simulink model "HFMA_4B_1_5_9_13"  (R2026b)
settings: Solver=FixedStepDiscrete  StopTime=stopTime  FixedStep=Ts
PreLoadFcn:
  | load('a_luts.mat')
values from neighbouring files (symbols this model uses):
  cosLUT = [1 1 1 1 1 1 1 1 1 1 1 1 ... (640 elements, 16x40)]    [iq_luts.mat]
  k_avg = 10    [Simulink_DOA_Test.m]    (also in collect_ranges.m; optimised_error_code.m)
  sinLUT = [0 0 0 0 0 0 0 0 0 0 0 0 ... (640 elements, 16x40)]    [iq_luts.mat]
  Ts = 1/8000    (= 0.000125)    [Simulink_DOA_Test.m]    (also in collect_ranges.m; optimised_error_code.m)
undefined symbols (not defined in the file or in its folder): a2_Im, a2_Re, a3_Im, a3_Re, NumBits1, NumBits2, Slope1, Slope2
libraries: hdlsllib x4, sl_signal_attributes x2
(part 2 of 6)

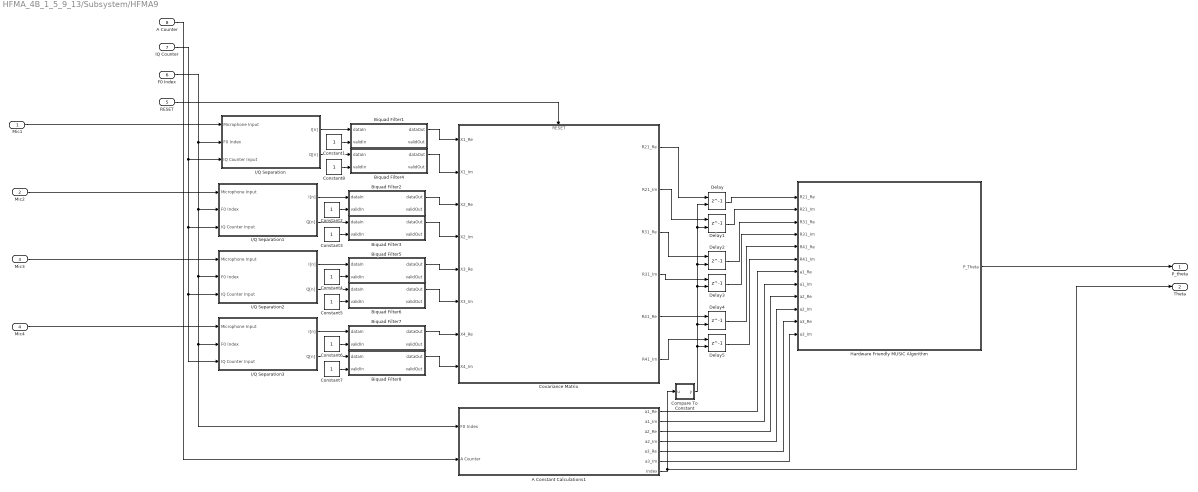
== system HFMA_4B_1_5_9_13/Subsystem/HFMA9 ==
  Mic1 : Inport
  Mic2 : Inport  Port=2
  Mic3 : Inport  Port=3
  Mic4 : Inport  Port=4
  RESET : Inport  Port=5
  F0 Index : Inport  Port=6
  IQ Counter : Inport  Port=7
  A Counter : Inport  Port=8
  A Constant Calculations1 : Subsystem
  Biquad Filter1 : Subsystem
  Biquad Filter2 : Subsystem
  Biquad Filter3 : Subsystem
  Biquad Filter4 : Subsystem
  Biquad Filter5 : Subsystem
  Biquad Filter6 : Subsystem
  Biquad Filter7 : Subsystem
  Biquad Filter8 : Subsystem
  Compare To Constant : Subsystem  mask(Compare To Constant){relop===, const=180, OutDataTypeStr=boolean, ZeroCross=on}
      mask prompts: relop "Simulink:masks:Operator_MP"; const "Simulink:masks:ConstantValue_MP"; OutDataTypeStr "Simulink:masks:OutputDataType_MP"; ZeroCross "Simulink:masks:EnableZerocrossingDetection_MP"
      mask help: Simulink:masks:CompareToConstant_MD
      mask init: same as HFMA_4B_1_5_9_13/Subsystem/HFMA1/Compare To Constant
      mask TypeOptions relop: == | ~= | < | <= | >= | >
      mask TypeOptions OutDataTypeStr: Simulink:masks:uint8 | Simulink:masks:boolean
      mask Callback ZeroCross: sl('zeroCrossEnable', gcbh);
      mask DialogControl relop Prompt: Operator:
      mask DialogControl const Prompt: Constant value:
      mask DialogControl OutDataTypeStr Prompt: Output data type:
      mask DialogControl ZeroCross Prompt: Enable zero-crossing detection
      mask Display: disp(str)
  Constant{1..8} (8 alike) : Constant  OutDataTypeStr=boolean
  Covariance Matrix : Subsystem
      settings: PortSchema="{\"entries\":[{\"content\":{\"sides\":[{\"content\":{\"connectorIds\":[\"In1\",\"In2\",\"In3\",\"In4\",\"In5\",\"In6\",\"In7\",\"In8\"]},\"type\":\"ConnectorPlacement.EquallySpacedRectSide\",\"uuid\":\"8604b8bd-6437-4f61-845f-68e8b5fac389\"},{\"content\":{\"connectorIds\":[\"Out1\",\"Out2\",\"Out3\",\"Out4\",\"Out5\",\"Out6\"],\"side\":\"RIGHT\"},\"type\":\"ConnectorPlacement.EquallySpacedRectSide\",\"uuid\":\"d39fd40c-d67e-46d5-b0a8-3014e1ecc186\"},{\"content\":{\"connectorIds\":[\"In9\"],\"side\":\"TOP\"},\"type\":\"ConnectorPlacement.EquallySpacedRectSide\",\"uuid\":\"4f74e432-20d9-4ae9-a889-27e37d930d6f\"},{\"content\":{\"side\":\"BOTTOM\"},\"type\":\"ConnectorPlacement.EquallySpacedRectSide\",\"uuid\":\"6d71da68-886d-48a5-a91d-56b84ddd4bf2\"}]},\"type\":\"ConnectorPlacement.EquallySpacedConnector\",\"uuid\":\"ca37f2c3-e85f-4529-98b4-a6b5e671d78f\"}],\"packageUris\":[\"http://schema.mathworks.com/mf0/Connector/R2020b\"],\"version\":\"1.0\"}"
  Delay{,1..5} (6 alike) : Delay  DelayLength=1  ShowEnablePort=on
      settings: InputPortMap=u0,e6
  Hardware Friendly MUSIC Algorithm : Subsystem
  I/Q Separation : Subsystem
  I/Q Separation1 : Subsystem
  I/Q Separation2 : Subsystem
  I/Q Separation3 : Subsystem
  P_theta : Outport
  Theta : Outport  Port=2
  wires:
  Covariance Matrix/2(R21_Im) -> Delay1/1
  Delay5/1 -> Hardware Friendly MUSIC Algorithm/6(R41_Im)
  Delay1/1 -> Hardware Friendly MUSIC Algorithm/2(R21_Im)
  A Constant Calculations1/3(a2_Re) -> Hardware Friendly MUSIC Algorithm/9(a2_Re)
  A Constant Calculations1/5(a3_Re) -> Hardware Friendly MUSIC Algorithm/11(a3_Re)
  Delay3/1 -> Hardware Friendly MUSIC Algorithm/4(R31_Im)
  Hardware Friendly MUSIC Algorithm/1(P_Theta) -> P_theta/1
  A Constant Calculations1/2(a1_Im) -> Hardware Friendly MUSIC Algorithm/8(a1_Im)
  Covariance Matrix/6(R41_Im) -> Delay5/1
  Delay4/1 -> Hardware Friendly MUSIC Algorithm/5(R41_Re)
  RESET/1 -> Covariance Matrix/9(RESET)
  Covariance Matrix/4(R31_Im) -> Delay3/1
  A Constant Calculations1/1(a1_Re) -> Hardware Friendly MUSIC Algorithm/7(a1_Re)
  Compare To Constant/1(y) -> Delay5/2, Delay/2, Delay1/2, Delay2/2, Delay3/2, Delay4/2
  Covariance Matrix/5(R41_Re) -> Delay4/1
  Delay/1 -> Hardware Friendly MUSIC Algorithm/1(R21_Re)
  A Constant Calculations1/4(a2_Im) -> Hardware Friendly MUSIC Algorithm/10(a2_Im)
  Delay2/1 -> Hardware Friendly MUSIC Algorithm/3(R31_Re)
  Covariance Matrix/1(R21_Re) -> Delay/1
  A Constant Calculations1/7(Index) -> Compare To Constant/1(u), Theta/1
  Covariance Matrix/3(R31_Re) -> Delay2/1
  A Constant Calculations1/6(a3_Im) -> Hardware Friendly MUSIC Algorithm/12(a3_Im)
  F0 Index/1 -> I/Q Separation1/2(F0 Index), I/Q Separation3/2(F0 Index), A Constant Calculations1/1(F0 Index), I/Q Separation2/2(F0 Index), I/Q Separation/2(F0 Index)
  IQ Counter/1 -> I/Q Separation3/3(IQ Counter Input), I/Q Separation2/3(IQ Counter Input), I/Q Separation1/3(IQ Counter Input), I/Q Separation/3(IQ Counter Input)
  Mic1/1 -> I/Q Separation/1(Microphone Input)
  Mic2/1 -> I/Q Separation1/1(Microphone Input)
  Mic3/1 -> I/Q Separation2/1(Microphone Input)
  Mic4/1 -> I/Q Separation3/1(Microphone Input)
  A Counter/1 -> A Constant Calculations1/2(A Counter)
  I/Q Separation/1(I[n]) -> Biquad Filter1/1(dataIn)
  Constant1/1 -> Biquad Filter1/2(validIn)
  Biquad Filter1/1(dataOut) -> Covariance Matrix/1(X1_Re)
  I/Q Separation1/1(I[n]) -> Biquad Filter2/1(dataIn)
  Constant2/1 -> Biquad Filter2/2(validIn)
  Biquad Filter2/1(dataOut) -> Covariance Matrix/3(X2_Re)
  I/Q Separation1/2(Q[n]) -> Biquad Filter3/1(dataIn)
  Constant3/1 -> Biquad Filter3/2(validIn)
  Biquad Filter3/1(dataOut) -> Covariance Matrix/4(X2_Im)
  I/Q Separation/2(Q[n]) -> Biquad Filter4/1(dataIn)
  Constant8/1 -> Biquad Filter4/2(validIn)
  Biquad Filter4/1(dataOut) -> Covariance Matrix/2(X1_Im)
  I/Q Separation2/1(I[n]) -> Biquad Filter5/1(dataIn)
  Constant4/1 -> Biquad Filter5/2(validIn)
  Biquad Filter5/1(dataOut) -> Covariance Matrix/5(X3_Re)
  I/Q Separation2/2(Q[n]) -> Biquad Filter6/1(dataIn)
  Constant5/1 -> Biquad Filter6/2(validIn)
  Biquad Filter6/1(dataOut) -> Covariance Matrix/6(X3_Im)
  I/Q Separation3/1(I[n]) -> Biquad Filter7/1(dataIn)
  Constant6/1 -> Biquad Filter7/2(validIn)
  Biquad Filter7/1(dataOut) -> Covariance Matrix/7(X4_Re)
  I/Q Separation3/2(Q[n]) -> Biquad Filter8/1(dataIn)
  Constant7/1 -> Biquad Filter8/2(validIn)
  Biquad Filter8/1(dataOut) -> Covariance Matrix/8(X4_Im)

== system HFMA_4B_1_5_9_13/Subsystem/IQ Counter ==
  Data Type Propagation : sl_signal_attributes/Data Type Propagation  PropDataTypeMode=Specify via dialog  PropDataType=uint(nbits)  IfRefDouble=double  IfRefSingle=single  IsSigned=IsSigned1 or IsSigned2  NumBitsBase=max([NumBits1 NumBits2])  NumBitsMult=1  NumBitsAdd=0  NumBitsAllowFinal=-1  PropScalingMode=Specify via dialog  PropScaling=1  ValuesUsedBestPrec=[5 -7]  SlopeBase=min([Slope1 Slope2])  SlopeMult=1  SlopeAdd=0  BiasBase=Bias1  BiasMult=1  BiasAdd=0
  Force to be scalar : SignalSpecification  DisableCoverage=on  Dimensions=1
  Increment Real World : hdlsllib/Math Operations/Increment Real World
  Output : UnitDelay  InitialCondition=0.0  SampleTime=tsamp
  Wrap To Zero : hdlsllib/Discontinuities/Wrap To Zero  Threshold=uplimit
  y : Outport
  wires:
  Increment Real World/1 -> Wrap To Zero/1
  Force to be scalar/1 -> Increment Real World/1
  Output/1 -> Force to be scalar/1, y/1
  Wrap To Zero/1 -> Output/1, Data Type Propagation/3, Data Type Propagation/2, Data Type Propagation/1

== system HFMA_4B_1_5_9_13/Subsystem/Max Theta Selector ==
  note: Latches the Output
  P_Theta : Inport
  Theta : Inport  Port=2
  RESET : Inport  Port=3
  Compare To Constant : Subsystem  mask(Compare To Constant){relop=<=, const=0, OutDataTypeStr=boolean, ZeroCross=on}
      mask prompts: relop "Simulink:masks:Operator_MP"; const "Simulink:masks:ConstantValue_MP"; OutDataTypeStr "Simulink:masks:OutputDataType_MP"; ZeroCross "Simulink:masks:EnableZerocrossingDetection_MP"
      mask help: Simulink:masks:CompareToConstant_MD
      mask init: same as HFMA_4B_1_5_9_13/Subsystem/HFMA1/Compare To Constant
      mask TypeOptions relop: == | ~= | < | <= | >= | >
      mask TypeOptions OutDataTypeStr: Simulink:masks:uint8 | Simulink:masks:boolean
      mask Callback ZeroCross: sl('zeroCrossEnable', gcbh);
      mask DialogControl relop Prompt: Operator:
      mask DialogControl const Prompt: Constant value:
      mask DialogControl OutDataTypeStr Prompt: Output data type:
      mask DialogControl ZeroCross Prompt: Enable zero-crossing detection
      mask Display: disp(str)
  Compare To Constant1 : Subsystem  mask(Compare To Constant){relop===, const=180, OutDataTypeStr=boolean, ZeroCross=on}
      mask prompts: relop "Simulink:masks:Operator_MP"; const "Simulink:masks:ConstantValue_MP"; OutDataTypeStr "Simulink:masks:OutputDataType_MP"; ZeroCross "Simulink:masks:EnableZerocrossingDetection_MP"
      mask help: Simulink:masks:CompareToConstant_MD
      mask init: same as HFMA_4B_1_5_9_13/Subsystem/HFMA1/Compare To Constant
      mask TypeOptions relop: == | ~= | < | <= | >= | >
      mask TypeOptions OutDataTypeStr: Simulink:masks:uint8 | Simulink:masks:boolean
      mask Callback ZeroCross: sl('zeroCrossEnable', gcbh);
      mask DialogControl relop Prompt: Operator:
      mask DialogControl const Prompt: Constant value:
      mask DialogControl OutDataTypeStr Prompt: Output data type:
      mask DialogControl ZeroCross Prompt: Enable zero-crossing detection
      mask Display: disp(str)
  Constant : Constant  Value=90  OutDataTypeStr=fixdt(0,18,11)
  Delay : Delay  DelayLength=1
  Delay1 : Delay  DelayLength=1
  Delay3 : Delay  DelayLength=1  ShowEnablePort=on
      settings: InputPortMap=u0,e6
  Logical Operator : Logic  Operator=OR  Inputs=3  AllPortsSameDT=off  OutDataTypeStr=boolean
  Relational Operator : RelationalOperator  Operator=>  OutDataTypeStr=boolean  RndMeth=Simplest  InputSameDT=off
  Subtract : Sum  Inputs=+-  OutDataTypeStr=fixdt(1,18,10)  SaturateOnIntegerOverflow=on
  Switch : Switch  Criteria=u2 ~= 0  SaturateOnIntegerOverflow=off  InputSameDT=off
  Switch1 : Switch  Criteria=u2 ~= 0  SaturateOnIntegerOverflow=off  InputSameDT=off
  Strongest Angle : Outport
  wires:
  Delay/1 -> Switch/3, Relational Operator/2
  Switch1/1 -> Delay1/1
  Switch/1 -> Delay/1
  Relational Operator/1 -> Logical Operator/1
  P_Theta/1 -> Switch/1, Relational Operator/1
  Theta/1 -> Compare To Constant1/1(u), Switch1/1, Compare To Constant/1(u)
  Constant/1 -> Subtract/2
  Subtract/1 -> Strongest Angle/1
  Compare To Constant/1(y) -> Logical Operator/3
  RESET/1 -> Logical Operator/2
  Logical Operator/1 -> Switch1/2, Switch/2
  Compare To Constant1/1(y) -> Delay3/2
  Delay1/1 -> Delay3/1, Switch1/3
  Delay3/1 -> Subtract/1

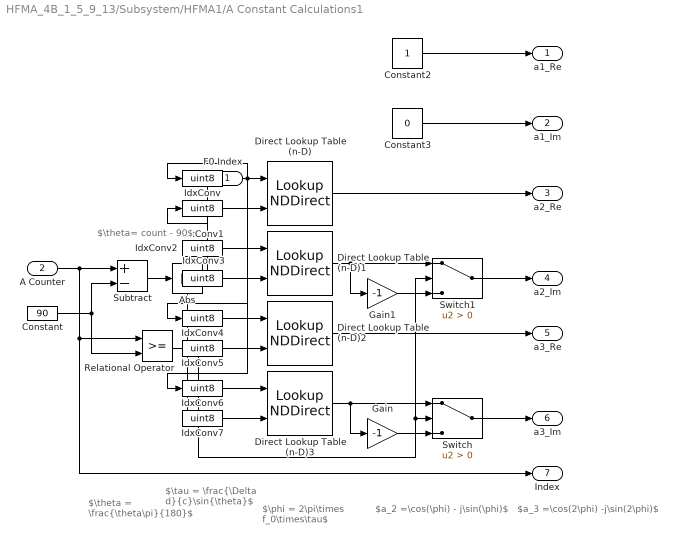
== system HFMA_4B_1_5_9_13/Subsystem/HFMA1/A Constant Calculations1 ==
  note: $\theta = \frac{\theta\pi}{180}$
  note: $\phi = 2\pi\times f_0\times\tau$
  note: $\tau = \frac{\Delta d}{c}\sin{\theta}$
  note: $\theta= count - 90$
  note: $a_2 =\cos(\phi) - j\sin(\phi)$
  note: $a_3 =\cos(2\phi) -j\sin(2\phi)$
  F0 Index : Inport
  A Counter : Inport  Port=2
  Abs : Abs  OutDataTypeStr=fixdt(1,18,0)  SaturateOnIntegerOverflow=off
  Constant : Constant  Value=90  OutDataTypeStr=fixdt(0,18,11)
  Constant2 : Constant  OutDataTypeStr=fixdt(0,18,17)
  Constant3 : Constant  Value=0  OutDataTypeStr=fixdt(1,18,4)
  Direct Lookup Table (n-D) : LookupNDDirect  Table=[a2_Re]  TableDataTypeStr=fixdt(1,18,16)
  Direct Lookup Table (n-D)1 : LookupNDDirect  Table=[a2_Im]  TableDataTypeStr=fixdt(1,18,17)
  Direct Lookup Table (n-D)2 : LookupNDDirect  Table=[a3_Re]  TableDataTypeStr=fixdt(1,18,16)
  Direct Lookup Table (n-D)3 : LookupNDDirect  Table=[a3_Im]  TableDataTypeStr=fixdt(1,18,17)
  Gain : Gain  Gain=-1  ParamDataTypeStr=fixdt(1,18,17)  OutDataTypeStr=fixdt(0,18,18)  SaturateOnIntegerOverflow=on
  Gain1 : Gain  Gain=-1  ParamDataTypeStr=fixdt(1,18,17)  OutDataTypeStr=fixdt(0,18,18)  SaturateOnIntegerOverflow=on
  IdxConv{,1..7} (8 alike) : DataTypeConversion  OutDataTypeStr=uint8  RndMeth=Floor
  Relational Operator : RelationalOperator  OutDataTypeStr=boolean  RndMeth=Simplest  InputSameDT=off
  Subtract : Sum  Inputs=+-  OutDataTypeStr=fixdt(1,18,0)  SaturateOnIntegerOverflow=on
  Switch : Switch  Criteria=u2 > Threshold  OutDataTypeStr=fixdt(1,18,17)  SaturateOnIntegerOverflow=off  InputSameDT=off
  Switch1 : Switch  Criteria=u2 > Threshold  OutDataTypeStr=fixdt(1,18,17)  SaturateOnIntegerOverflow=off  InputSameDT=off
  a1_Re : Outport
  a1_Im : Outport  Port=2
  a2_Re : Outport  Port=3
  a2_Im : Outport  Port=4
  a3_Re : Outport  Port=5
  a3_Im : Outport  Port=6
  Index : Outport  Port=7
  wires:
  A Counter/1 -> Relational Operator/1, Index/1, Subtract/1
  Constant/1 -> Subtract/2, Relational Operator/2
  Constant2/1 -> a1_Re/1
  Constant3/1 -> a1_Im/1
  F0 Index/1 -> IdxConv/1, IdxConv2/1, IdxConv4/1, IdxConv6/1
  Subtract/1 -> Abs/1
  Direct Lookup Table (n-D)/1 -> a2_Re/1
  Direct Lookup Table (n-D)2/1 -> a3_Re/1
  Direct Lookup Table (n-D)1/1 -> Switch1/1, Gain1/1
  Direct Lookup Table (n-D)3/1 -> Switch/1, Gain/1
  Gain/1 -> Switch/3
  Gain1/1 -> Switch1/3
  Relational Operator/1 -> Switch/2, Switch1/2
  Switch/1 -> a3_Im/1
  Switch1/1 -> a2_Im/1
  Abs/1 -> IdxConv1/1, IdxConv3/1, IdxConv5/1, IdxConv7/1
  IdxConv/1 -> Direct Lookup Table (n-D)/1
  IdxConv1/1 -> Direct Lookup Table (n-D)/2
  IdxConv2/1 -> Direct Lookup Table (n-D)1/1
  IdxConv3/1 -> Direct Lookup Table (n-D)1/2
  IdxConv4/1 -> Direct Lookup Table (n-D)2/1
  IdxConv5/1 -> Direct Lookup Table (n-D)2/2
  IdxConv6/1 -> Direct Lookup Table (n-D)3/1
  IdxConv7/1 -> Direct Lookup Table (n-D)3/2

== system HFMA_4B_1_5_9_13/Subsystem/HFMA1/Biquad Filter1 ==
  dataIn : Inport
  validIn : Inport  Port=2
  D1_1 : Delay  DelayLength=1  InitialCondition=0
  D1_2 : Delay  DelayLength=1  InitialCondition=0
  D2_1 : Delay  DelayLength=1  InitialCondition=0
  D2_2 : Delay  DelayLength=1  InitialCondition=0
  Q_1 : DataTypeConversion  OutDataTypeStr=fixdt(1,18,16)  RndMeth=Floor
  Q_2 : DataTypeConversion  OutDataTypeStr=fixdt(1,18,16)  RndMeth=Floor
  S0_1 : Sum  OutDataTypeStr=fixdt(1,40,30)  SaturateOnIntegerOverflow=on
  S0_2 : Sum  OutDataTypeStr=fixdt(1,40,30)  SaturateOnIntegerOverflow=on
  S1_1 : Sum  Inputs=+++  OutDataTypeStr=fixdt(1,40,30)  SaturateOnIntegerOverflow=on
  S1_2 : Sum  Inputs=+++  OutDataTypeStr=fixdt(1,40,30)  SaturateOnIntegerOverflow=on
  S2_1 : Sum  OutDataTypeStr=fixdt(1,40,30)  SaturateOnIntegerOverflow=on
  S2_2 : Sum  OutDataTypeStr=fixdt(1,40,30)  SaturateOnIntegerOverflow=on
  b0_1 : Gain  Gain=0.0011721199932606119  ParamDataTypeStr=fixdt(1,18,26)  OutDataTypeStr=fixdt(1,40,30)  SaturateOnIntegerOverflow=on
  b0_2 : Gain  Gain=0.0012157429617273841  ParamDataTypeStr=fixdt(1,18,26)  OutDataTypeStr=fixdt(1,40,30)  SaturateOnIntegerOverflow=on
  b1_1 : Gain  Gain=0.0023442399865212238  ParamDataTypeStr=fixdt(1,18,25)  OutDataTypeStr=fixdt(1,40,30)  SaturateOnIntegerOverflow=on
  b1_2 : Gain  Gain=0.0024314859234547681  ParamDataTypeStr=fixdt(1,18,25)  OutDataTypeStr=fixdt(1,40,30)  SaturateOnIntegerOverflow=on
  b2_1 : Gain  Gain=0.0011721199932606119  ParamDataTypeStr=fixdt(1,18,26)  OutDataTypeStr=fixdt(1,40,30)  SaturateOnIntegerOverflow=on
  b2_2 : Gain  Gain=0.0012157429617273841  ParamDataTypeStr=fixdt(1,18,26)  OutDataTypeStr=fixdt(1,40,30)  SaturateOnIntegerOverflow=on
  na1_1 : Gain  Gain=1.8728036090138058  ParamDataTypeStr=fixdt(1,18,16)  OutDataTypeStr=fixdt(1,40,30)  SaturateOnIntegerOverflow=on
  na1_2 : Gain  Gain=1.942504026420016  ParamDataTypeStr=fixdt(1,18,16)  OutDataTypeStr=fixdt(1,40,30)  SaturateOnIntegerOverflow=on
  na2_1 : Gain  Gain=-0.87749208898684827  ParamDataTypeStr=fixdt(1,18,17)  OutDataTypeStr=fixdt(1,40,30)  SaturateOnIntegerOverflow=on
  na2_2 : Gain  Gain=-0.9473669982669255  ParamDataTypeStr=fixdt(1,18,17)  OutDataTypeStr=fixdt(1,40,30)  SaturateOnIntegerOverflow=on
  dataOut : Outport
  validOut : Outport  Port=2
  wires:
  S2_2/1 -> D2_2/1
  S1_2/1 -> D1_2/1
  na2_2/1 -> S2_2/2
  b2_2/1 -> S2_2/1
  D2_2/1 -> S1_2/3
  na1_2/1 -> S1_2/2
  b1_2/1 -> S1_2/1
  Q_2/1 -> dataOut/1, na2_2/1, na1_2/1
  S0_2/1 -> Q_2/1
  D1_2/1 -> S0_2/2
  b0_2/1 -> S0_2/1
  S2_1/1 -> D2_1/1
  S1_1/1 -> D1_1/1
  na2_1/1 -> S2_1/2
  b2_1/1 -> S2_1/1
  D2_1/1 -> S1_1/3
  na1_1/1 -> S1_1/2
  b1_1/1 -> S1_1/1
  Q_1/1 -> b2_2/1, b1_2/1, b0_2/1, na2_1/1, na1_1/1
  S0_1/1 -> Q_1/1
  D1_1/1 -> S0_1/2
  b0_1/1 -> S0_1/1
  dataIn/1 -> b2_1/1, b1_1/1, b0_1/1
  validIn/1 -> validOut/1

== system HFMA_4B_1_5_9_13/Subsystem/HFMA1/Biquad Filter2 ==
  dataIn : Inport
  validIn : Inport  Port=2
  D1_1 : Delay  DelayLength=1  InitialCondition=0
  D1_2 : Delay  DelayLength=1  InitialCondition=0
  D2_1 : Delay  DelayLength=1  InitialCondition=0
  D2_2 : Delay  DelayLength=1  InitialCondition=0
  Q_1 : DataTypeConversion  OutDataTypeStr=fixdt(1,18,16)  RndMeth=Floor
  Q_2 : DataTypeConversion  OutDataTypeStr=fixdt(1,18,16)  RndMeth=Floor
  S0_1 : Sum  OutDataTypeStr=fixdt(1,40,30)  SaturateOnIntegerOverflow=on
  S0_2 : Sum  OutDataTypeStr=fixdt(1,40,30)  SaturateOnIntegerOverflow=on
  S1_1 : Sum  Inputs=+++  OutDataTypeStr=fixdt(1,40,30)  SaturateOnIntegerOverflow=on
  S1_2 : Sum  Inputs=+++  OutDataTypeStr=fixdt(1,40,30)  SaturateOnIntegerOverflow=on
  S2_1 : Sum  OutDataTypeStr=fixdt(1,40,30)  SaturateOnIntegerOverflow=on
  S2_2 : Sum  OutDataTypeStr=fixdt(1,40,30)  SaturateOnIntegerOverflow=on
  b0_1 : Gain  Gain=0.0011721199932606119  ParamDataTypeStr=fixdt(1,18,26)  OutDataTypeStr=fixdt(1,40,30)  SaturateOnIntegerOverflow=on
  b0_2 : Gain  Gain=0.0012157429617273841  ParamDataTypeStr=fixdt(1,18,26)  OutDataTypeStr=fixdt(1,40,30)  SaturateOnIntegerOverflow=on
  b1_1 : Gain  Gain=0.0023442399865212238  ParamDataTypeStr=fixdt(1,18,25)  OutDataTypeStr=fixdt(1,40,30)  SaturateOnIntegerOverflow=on
  b1_2 : Gain  Gain=0.0024314859234547681  ParamDataTypeStr=fixdt(1,18,25)  OutDataTypeStr=fixdt(1,40,30)  SaturateOnIntegerOverflow=on
  b2_1 : Gain  Gain=0.0011721199932606119  ParamDataTypeStr=fixdt(1,18,26)  OutDataTypeStr=fixdt(1,40,30)  SaturateOnIntegerOverflow=on
  b2_2 : Gain  Gain=0.0012157429617273841  ParamDataTypeStr=fixdt(1,18,26)  OutDataTypeStr=fixdt(1,40,30)  SaturateOnIntegerOverflow=on
  na1_1 : Gain  Gain=1.8728036090138058  ParamDataTypeStr=fixdt(1,18,16)  OutDataTypeStr=fixdt(1,40,30)  SaturateOnIntegerOverflow=on
  na1_2 : Gain  Gain=1.942504026420016  ParamDataTypeStr=fixdt(1,18,16)  OutDataTypeStr=fixdt(1,40,30)  SaturateOnIntegerOverflow=on
  na2_1 : Gain  Gain=-0.87749208898684827  ParamDataTypeStr=fixdt(1,18,17)  OutDataTypeStr=fixdt(1,40,30)  SaturateOnIntegerOverflow=on
  na2_2 : Gain  Gain=-0.9473669982669255  ParamDataTypeStr=fixdt(1,18,17)  OutDataTypeStr=fixdt(1,40,30)  SaturateOnIntegerOverflow=on
  dataOut : Outport
  validOut : Outport  Port=2
  wires:
  S2_2/1 -> D2_2/1
  S1_2/1 -> D1_2/1
  na2_2/1 -> S2_2/2
  b2_2/1 -> S2_2/1
  D2_2/1 -> S1_2/3
  na1_2/1 -> S1_2/2
  b1_2/1 -> S1_2/1
  Q_2/1 -> dataOut/1, na2_2/1, na1_2/1
  S0_2/1 -> Q_2/1
  D1_2/1 -> S0_2/2
  b0_2/1 -> S0_2/1
  S2_1/1 -> D2_1/1
  S1_1/1 -> D1_1/1
  na2_1/1 -> S2_1/2
  b2_1/1 -> S2_1/1
  D2_1/1 -> S1_1/3
  na1_1/1 -> S1_1/2
  b1_1/1 -> S1_1/1
  Q_1/1 -> b2_2/1, b1_2/1, b0_2/1, na2_1/1, na1_1/1
  S0_1/1 -> Q_1/1
  D1_1/1 -> S0_1/2
  b0_1/1 -> S0_1/1
  dataIn/1 -> b2_1/1, b1_1/1, b0_1/1
  validIn/1 -> validOut/1

== system HFMA_4B_1_5_9_13/Subsystem/HFMA1/Biquad Filter3 ==
  dataIn : Inport
  validIn : Inport  Port=2
  D1_1 : Delay  DelayLength=1  InitialCondition=0
  D1_2 : Delay  DelayLength=1  InitialCondition=0
  D2_1 : Delay  DelayLength=1  InitialCondition=0
  D2_2 : Delay  DelayLength=1  InitialCondition=0
  Q_1 : DataTypeConversion  OutDataTypeStr=fixdt(1,18,16)  RndMeth=Floor
  Q_2 : DataTypeConversion  OutDataTypeStr=fixdt(1,18,16)  RndMeth=Floor
  S0_1 : Sum  OutDataTypeStr=fixdt(1,40,30)  SaturateOnIntegerOverflow=on
  S0_2 : Sum  OutDataTypeStr=fixdt(1,40,30)  SaturateOnIntegerOverflow=on
  S1_1 : Sum  Inputs=+++  OutDataTypeStr=fixdt(1,40,30)  SaturateOnIntegerOverflow=on
  S1_2 : Sum  Inputs=+++  OutDataTypeStr=fixdt(1,40,30)  SaturateOnIntegerOverflow=on
  S2_1 : Sum  OutDataTypeStr=fixdt(1,40,30)  SaturateOnIntegerOverflow=on
  S2_2 : Sum  OutDataTypeStr=fixdt(1,40,30)  SaturateOnIntegerOverflow=on
  b0_1 : Gain  Gain=0.0011721199932606119  ParamDataTypeStr=fixdt(1,18,26)  OutDataTypeStr=fixdt(1,40,30)  SaturateOnIntegerOverflow=on
  b0_2 : Gain  Gain=0.0012157429617273841  ParamDataTypeStr=fixdt(1,18,26)  OutDataTypeStr=fixdt(1,40,30)  SaturateOnIntegerOverflow=on
  b1_1 : Gain  Gain=0.0023442399865212238  ParamDataTypeStr=fixdt(1,18,25)  OutDataTypeStr=fixdt(1,40,30)  SaturateOnIntegerOverflow=on
  b1_2 : Gain  Gain=0.0024314859234547681  ParamDataTypeStr=fixdt(1,18,25)  OutDataTypeStr=fixdt(1,40,30)  SaturateOnIntegerOverflow=on
  b2_1 : Gain  Gain=0.0011721199932606119  ParamDataTypeStr=fixdt(1,18,26)  OutDataTypeStr=fixdt(1,40,30)  SaturateOnIntegerOverflow=on
  b2_2 : Gain  Gain=0.0012157429617273841  ParamDataTypeStr=fixdt(1,18,26)  OutDataTypeStr=fixdt(1,40,30)  SaturateOnIntegerOverflow=on
  na1_1 : Gain  Gain=1.8728036090138058  ParamDataTypeStr=fixdt(1,18,16)  OutDataTypeStr=fixdt(1,40,30)  SaturateOnIntegerOverflow=on
  na1_2 : Gain  Gain=1.942504026420016  ParamDataTypeStr=fixdt(1,18,16)  OutDataTypeStr=fixdt(1,40,30)  SaturateOnIntegerOverflow=on
  na2_1 : Gain  Gain=-0.87749208898684827  ParamDataTypeStr=fixdt(1,18,17)  OutDataTypeStr=fixdt(1,40,30)  SaturateOnIntegerOverflow=on
  na2_2 : Gain  Gain=-0.9473669982669255  ParamDataTypeStr=fixdt(1,18,17)  OutDataTypeStr=fixdt(1,40,30)  SaturateOnIntegerOverflow=on
  dataOut : Outport
  validOut : Outport  Port=2
  wires:
  S2_2/1 -> D2_2/1
  S1_2/1 -> D1_2/1
  na2_2/1 -> S2_2/2
  b2_2/1 -> S2_2/1
  D2_2/1 -> S1_2/3
  na1_2/1 -> S1_2/2
  b1_2/1 -> S1_2/1
  Q_2/1 -> dataOut/1, na2_2/1, na1_2/1
  S0_2/1 -> Q_2/1
  D1_2/1 -> S0_2/2
  b0_2/1 -> S0_2/1
  S2_1/1 -> D2_1/1
  S1_1/1 -> D1_1/1
  na2_1/1 -> S2_1/2
  b2_1/1 -> S2_1/1
  D2_1/1 -> S1_1/3
  na1_1/1 -> S1_1/2
  b1_1/1 -> S1_1/1
  Q_1/1 -> b2_2/1, b1_2/1, b0_2/1, na2_1/1, na1_1/1
  S0_1/1 -> Q_1/1
  D1_1/1 -> S0_1/2
  b0_1/1 -> S0_1/1
  dataIn/1 -> b2_1/1, b1_1/1, b0_1/1
  validIn/1 -> validOut/1

== system HFMA_4B_1_5_9_13/Subsystem/HFMA1/Biquad Filter4 ==
  dataIn : Inport
  validIn : Inport  Port=2
  D1_1 : Delay  DelayLength=1  InitialCondition=0
  D1_2 : Delay  DelayLength=1  InitialCondition=0
  D2_1 : Delay  DelayLength=1  InitialCondition=0
  D2_2 : Delay  DelayLength=1  InitialCondition=0
  Q_1 : DataTypeConversion  OutDataTypeStr=fixdt(1,18,16)  RndMeth=Floor
  Q_2 : DataTypeConversion  OutDataTypeStr=fixdt(1,18,16)  RndMeth=Floor
  S0_1 : Sum  OutDataTypeStr=fixdt(1,40,30)  SaturateOnIntegerOverflow=on
  S0_2 : Sum  OutDataTypeStr=fixdt(1,40,30)  SaturateOnIntegerOverflow=on
  S1_1 : Sum  Inputs=+++  OutDataTypeStr=fixdt(1,40,30)  SaturateOnIntegerOverflow=on
  S1_2 : Sum  Inputs=+++  OutDataTypeStr=fixdt(1,40,30)  SaturateOnIntegerOverflow=on
  S2_1 : Sum  OutDataTypeStr=fixdt(1,40,30)  SaturateOnIntegerOverflow=on
  S2_2 : Sum  OutDataTypeStr=fixdt(1,40,30)  SaturateOnIntegerOverflow=on
  b0_1 : Gain  Gain=0.0011721199932606119  ParamDataTypeStr=fixdt(1,18,26)  OutDataTypeStr=fixdt(1,40,30)  SaturateOnIntegerOverflow=on
  b0_2 : Gain  Gain=0.0012157429617273841  ParamDataTypeStr=fixdt(1,18,26)  OutDataTypeStr=fixdt(1,40,30)  SaturateOnIntegerOverflow=on
  b1_1 : Gain  Gain=0.0023442399865212238  ParamDataTypeStr=fixdt(1,18,25)  OutDataTypeStr=fixdt(1,40,30)  SaturateOnIntegerOverflow=on
  b1_2 : Gain  Gain=0.0024314859234547681  ParamDataTypeStr=fixdt(1,18,25)  OutDataTypeStr=fixdt(1,40,30)  SaturateOnIntegerOverflow=on
  b2_1 : Gain  Gain=0.0011721199932606119  ParamDataTypeStr=fixdt(1,18,26)  OutDataTypeStr=fixdt(1,40,30)  SaturateOnIntegerOverflow=on
  b2_2 : Gain  Gain=0.0012157429617273841  ParamDataTypeStr=fixdt(1,18,26)  OutDataTypeStr=fixdt(1,40,30)  SaturateOnIntegerOverflow=on
  na1_1 : Gain  Gain=1.8728036090138058  ParamDataTypeStr=fixdt(1,18,16)  OutDataTypeStr=fixdt(1,40,30)  SaturateOnIntegerOverflow=on
  na1_2 : Gain  Gain=1.942504026420016  ParamDataTypeStr=fixdt(1,18,16)  OutDataTypeStr=fixdt(1,40,30)  SaturateOnIntegerOverflow=on
  na2_1 : Gain  Gain=-0.87749208898684827  ParamDataTypeStr=fixdt(1,18,17)  OutDataTypeStr=fixdt(1,40,30)  SaturateOnIntegerOverflow=on
  na2_2 : Gain  Gain=-0.9473669982669255  ParamDataTypeStr=fixdt(1,18,17)  OutDataTypeStr=fixdt(1,40,30)  SaturateOnIntegerOverflow=on
  dataOut : Outport
  validOut : Outport  Port=2
  wires:
  S2_2/1 -> D2_2/1
  S1_2/1 -> D1_2/1
  na2_2/1 -> S2_2/2
  b2_2/1 -> S2_2/1
  D2_2/1 -> S1_2/3
  na1_2/1 -> S1_2/2
  b1_2/1 -> S1_2/1
  Q_2/1 -> dataOut/1, na2_2/1, na1_2/1
  S0_2/1 -> Q_2/1
  D1_2/1 -> S0_2/2
  b0_2/1 -> S0_2/1
  S2_1/1 -> D2_1/1
  S1_1/1 -> D1_1/1
  na2_1/1 -> S2_1/2
  b2_1/1 -> S2_1/1
  D2_1/1 -> S1_1/3
  na1_1/1 -> S1_1/2
  b1_1/1 -> S1_1/1
  Q_1/1 -> b2_2/1, b1_2/1, b0_2/1, na2_1/1, na1_1/1
  S0_1/1 -> Q_1/1
  D1_1/1 -> S0_1/2
  b0_1/1 -> S0_1/1
  dataIn/1 -> b2_1/1, b1_1/1, b0_1/1
  validIn/1 -> validOut/1

== system HFMA_4B_1_5_9_13/Subsystem/HFMA1/Biquad Filter5 ==
  dataIn : Inport
  validIn : Inport  Port=2
  D1_1 : Delay  DelayLength=1  InitialCondition=0
  D1_2 : Delay  DelayLength=1  InitialCondition=0
  D2_1 : Delay  DelayLength=1  InitialCondition=0
  D2_2 : Delay  DelayLength=1  InitialCondition=0
  Q_1 : DataTypeConversion  OutDataTypeStr=fixdt(1,18,16)  RndMeth=Floor
  Q_2 : DataTypeConversion  OutDataTypeStr=fixdt(1,18,16)  RndMeth=Floor
  S0_1 : Sum  OutDataTypeStr=fixdt(1,40,30)  SaturateOnIntegerOverflow=on
  S0_2 : Sum  OutDataTypeStr=fixdt(1,40,30)  SaturateOnIntegerOverflow=on
  S1_1 : Sum  Inputs=+++  OutDataTypeStr=fixdt(1,40,30)  SaturateOnIntegerOverflow=on
  S1_2 : Sum  Inputs=+++  OutDataTypeStr=fixdt(1,40,30)  SaturateOnIntegerOverflow=on
  S2_1 : Sum  OutDataTypeStr=fixdt(1,40,30)  SaturateOnIntegerOverflow=on
  S2_2 : Sum  OutDataTypeStr=fixdt(1,40,30)  SaturateOnIntegerOverflow=on
  b0_1 : Gain  Gain=0.0011721199932606119  ParamDataTypeStr=fixdt(1,18,26)  OutDataTypeStr=fixdt(1,40,30)  SaturateOnIntegerOverflow=on
  b0_2 : Gain  Gain=0.0012157429617273841  ParamDataTypeStr=fixdt(1,18,26)  OutDataTypeStr=fixdt(1,40,30)  SaturateOnIntegerOverflow=on
  b1_1 : Gain  Gain=0.0023442399865212238  ParamDataTypeStr=fixdt(1,18,25)  OutDataTypeStr=fixdt(1,40,30)  SaturateOnIntegerOverflow=on
  b1_2 : Gain  Gain=0.0024314859234547681  ParamDataTypeStr=fixdt(1,18,25)  OutDataTypeStr=fixdt(1,40,30)  SaturateOnIntegerOverflow=on
  b2_1 : Gain  Gain=0.0011721199932606119  ParamDataTypeStr=fixdt(1,18,26)  OutDataTypeStr=fixdt(1,40,30)  SaturateOnIntegerOverflow=on
  b2_2 : Gain  Gain=0.0012157429617273841  ParamDataTypeStr=fixdt(1,18,26)  OutDataTypeStr=fixdt(1,40,30)  SaturateOnIntegerOverflow=on
  na1_1 : Gain  Gain=1.8728036090138058  ParamDataTypeStr=fixdt(1,18,16)  OutDataTypeStr=fixdt(1,40,30)  SaturateOnIntegerOverflow=on
  na1_2 : Gain  Gain=1.942504026420016  ParamDataTypeStr=fixdt(1,18,16)  OutDataTypeStr=fixdt(1,40,30)  SaturateOnIntegerOverflow=on
  na2_1 : Gain  Gain=-0.87749208898684827  ParamDataTypeStr=fixdt(1,18,17)  OutDataTypeStr=fixdt(1,40,30)  SaturateOnIntegerOverflow=on
  na2_2 : Gain  Gain=-0.9473669982669255  ParamDataTypeStr=fixdt(1,18,17)  OutDataTypeStr=fixdt(1,40,30)  SaturateOnIntegerOverflow=on
  dataOut : Outport
  validOut : Outport  Port=2
  wires:
  S2_2/1 -> D2_2/1
  S1_2/1 -> D1_2/1
  na2_2/1 -> S2_2/2
  b2_2/1 -> S2_2/1
  D2_2/1 -> S1_2/3
  na1_2/1 -> S1_2/2
  b1_2/1 -> S1_2/1
  Q_2/1 -> dataOut/1, na2_2/1, na1_2/1
  S0_2/1 -> Q_2/1
  D1_2/1 -> S0_2/2
  b0_2/1 -> S0_2/1
  S2_1/1 -> D2_1/1
  S1_1/1 -> D1_1/1
  na2_1/1 -> S2_1/2
  b2_1/1 -> S2_1/1
  D2_1/1 -> S1_1/3
  na1_1/1 -> S1_1/2
  b1_1/1 -> S1_1/1
  Q_1/1 -> b2_2/1, b1_2/1, b0_2/1, na2_1/1, na1_1/1
  S0_1/1 -> Q_1/1
  D1_1/1 -> S0_1/2
  b0_1/1 -> S0_1/1
  dataIn/1 -> b2_1/1, b1_1/1, b0_1/1
  validIn/1 -> validOut/1

== system HFMA_4B_1_5_9_13/Subsystem/HFMA1/Biquad Filter6 ==
  dataIn : Inport
  validIn : Inport  Port=2
  D1_1 : Delay  DelayLength=1  InitialCondition=0
  D1_2 : Delay  DelayLength=1  InitialCondition=0
  D2_1 : Delay  DelayLength=1  InitialCondition=0
  D2_2 : Delay  DelayLength=1  InitialCondition=0
  Q_1 : DataTypeConversion  OutDataTypeStr=fixdt(1,18,16)  RndMeth=Floor
  Q_2 : DataTypeConversion  OutDataTypeStr=fixdt(1,18,16)  RndMeth=Floor
  S0_1 : Sum  OutDataTypeStr=fixdt(1,40,30)  SaturateOnIntegerOverflow=on
  S0_2 : Sum  OutDataTypeStr=fixdt(1,40,30)  SaturateOnIntegerOverflow=on
  S1_1 : Sum  Inputs=+++  OutDataTypeStr=fixdt(1,40,30)  SaturateOnIntegerOverflow=on
  S1_2 : Sum  Inputs=+++  OutDataTypeStr=fixdt(1,40,30)  SaturateOnIntegerOverflow=on
  S2_1 : Sum  OutDataTypeStr=fixdt(1,40,30)  SaturateOnIntegerOverflow=on
  S2_2 : Sum  OutDataTypeStr=fixdt(1,40,30)  SaturateOnIntegerOverflow=on
  b0_1 : Gain  Gain=0.0011721199932606119  ParamDataTypeStr=fixdt(1,18,26)  OutDataTypeStr=fixdt(1,40,30)  SaturateOnIntegerOverflow=on
  b0_2 : Gain  Gain=0.0012157429617273841  ParamDataTypeStr=fixdt(1,18,26)  OutDataTypeStr=fixdt(1,40,30)  SaturateOnIntegerOverflow=on
  b1_1 : Gain  Gain=0.0023442399865212238  ParamDataTypeStr=fixdt(1,18,25)  OutDataTypeStr=fixdt(1,40,30)  SaturateOnIntegerOverflow=on
  b1_2 : Gain  Gain=0.0024314859234547681  ParamDataTypeStr=fixdt(1,18,25)  OutDataTypeStr=fixdt(1,40,30)  SaturateOnIntegerOverflow=on
  b2_1 : Gain  Gain=0.0011721199932606119  ParamDataTypeStr=fixdt(1,18,26)  OutDataTypeStr=fixdt(1,40,30)  SaturateOnIntegerOverflow=on
  b2_2 : Gain  Gain=0.0012157429617273841  ParamDataTypeStr=fixdt(1,18,26)  OutDataTypeStr=fixdt(1,40,30)  SaturateOnIntegerOverflow=on
  na1_1 : Gain  Gain=1.8728036090138058  ParamDataTypeStr=fixdt(1,18,16)  OutDataTypeStr=fixdt(1,40,30)  SaturateOnIntegerOverflow=on
  na1_2 : Gain  Gain=1.942504026420016  ParamDataTypeStr=fixdt(1,18,16)  OutDataTypeStr=fixdt(1,40,30)  SaturateOnIntegerOverflow=on
  na2_1 : Gain  Gain=-0.87749208898684827  ParamDataTypeStr=fixdt(1,18,17)  OutDataTypeStr=fixdt(1,40,30)  SaturateOnIntegerOverflow=on
  na2_2 : Gain  Gain=-0.9473669982669255  ParamDataTypeStr=fixdt(1,18,17)  OutDataTypeStr=fixdt(1,40,30)  SaturateOnIntegerOverflow=on
  dataOut : Outport
  validOut : Outport  Port=2
  wires:
  S2_2/1 -> D2_2/1
  S1_2/1 -> D1_2/1
  na2_2/1 -> S2_2/2
  b2_2/1 -> S2_2/1
  D2_2/1 -> S1_2/3
  na1_2/1 -> S1_2/2
  b1_2/1 -> S1_2/1
  Q_2/1 -> dataOut/1, na2_2/1, na1_2/1
  S0_2/1 -> Q_2/1
  D1_2/1 -> S0_2/2
  b0_2/1 -> S0_2/1
  S2_1/1 -> D2_1/1
  S1_1/1 -> D1_1/1
  na2_1/1 -> S2_1/2
  b2_1/1 -> S2_1/1
  D2_1/1 -> S1_1/3
  na1_1/1 -> S1_1/2
  b1_1/1 -> S1_1/1
  Q_1/1 -> b2_2/1, b1_2/1, b0_2/1, na2_1/1, na1_1/1
  S0_1/1 -> Q_1/1
  D1_1/1 -> S0_1/2
  b0_1/1 -> S0_1/1
  dataIn/1 -> b2_1/1, b1_1/1, b0_1/1
  validIn/1 -> validOut/1

== system HFMA_4B_1_5_9_13/Subsystem/HFMA1/Biquad Filter7 ==
  dataIn : Inport
  validIn : Inport  Port=2
  D1_1 : Delay  DelayLength=1  InitialCondition=0
  D1_2 : Delay  DelayLength=1  InitialCondition=0
  D2_1 : Delay  DelayLength=1  InitialCondition=0
  D2_2 : Delay  DelayLength=1  InitialCondition=0
  Q_1 : DataTypeConversion  OutDataTypeStr=fixdt(1,18,16)  RndMeth=Floor
  Q_2 : DataTypeConversion  OutDataTypeStr=fixdt(1,18,16)  RndMeth=Floor
  S0_1 : Sum  OutDataTypeStr=fixdt(1,40,30)  SaturateOnIntegerOverflow=on
  S0_2 : Sum  OutDataTypeStr=fixdt(1,40,30)  SaturateOnIntegerOverflow=on
  S1_1 : Sum  Inputs=+++  OutDataTypeStr=fixdt(1,40,30)  SaturateOnIntegerOverflow=on
  S1_2 : Sum  Inputs=+++  OutDataTypeStr=fixdt(1,40,30)  SaturateOnIntegerOverflow=on
  S2_1 : Sum  OutDataTypeStr=fixdt(1,40,30)  SaturateOnIntegerOverflow=on
  S2_2 : Sum  OutDataTypeStr=fixdt(1,40,30)  SaturateOnIntegerOverflow=on
  b0_1 : Gain  Gain=0.0011721199932606119  ParamDataTypeStr=fixdt(1,18,26)  OutDataTypeStr=fixdt(1,40,30)  SaturateOnIntegerOverflow=on
  b0_2 : Gain  Gain=0.0012157429617273841  ParamDataTypeStr=fixdt(1,18,26)  OutDataTypeStr=fixdt(1,40,30)  SaturateOnIntegerOverflow=on
  b1_1 : Gain  Gain=0.0023442399865212238  ParamDataTypeStr=fixdt(1,18,25)  OutDataTypeStr=fixdt(1,40,30)  SaturateOnIntegerOverflow=on
  b1_2 : Gain  Gain=0.0024314859234547681  ParamDataTypeStr=fixdt(1,18,25)  OutDataTypeStr=fixdt(1,40,30)  SaturateOnIntegerOverflow=on
  b2_1 : Gain  Gain=0.0011721199932606119  ParamDataTypeStr=fixdt(1,18,26)  OutDataTypeStr=fixdt(1,40,30)  SaturateOnIntegerOverflow=on
  b2_2 : Gain  Gain=0.0012157429617273841  ParamDataTypeStr=fixdt(1,18,26)  OutDataTypeStr=fixdt(1,40,30)  SaturateOnIntegerOverflow=on
  na1_1 : Gain  Gain=1.8728036090138058  ParamDataTypeStr=fixdt(1,18,16)  OutDataTypeStr=fixdt(1,40,30)  SaturateOnIntegerOverflow=on
  na1_2 : Gain  Gain=1.942504026420016  ParamDataTypeStr=fixdt(1,18,16)  OutDataTypeStr=fixdt(1,40,30)  SaturateOnIntegerOverflow=on
  na2_1 : Gain  Gain=-0.87749208898684827  ParamDataTypeStr=fixdt(1,18,17)  OutDataTypeStr=fixdt(1,40,30)  SaturateOnIntegerOverflow=on
  na2_2 : Gain  Gain=-0.9473669982669255  ParamDataTypeStr=fixdt(1,18,17)  OutDataTypeStr=fixdt(1,40,30)  SaturateOnIntegerOverflow=on
  dataOut : Outport
  validOut : Outport  Port=2
  wires:
  S2_2/1 -> D2_2/1
  S1_2/1 -> D1_2/1
  na2_2/1 -> S2_2/2
  b2_2/1 -> S2_2/1
  D2_2/1 -> S1_2/3
  na1_2/1 -> S1_2/2
  b1_2/1 -> S1_2/1
  Q_2/1 -> dataOut/1, na2_2/1, na1_2/1
  S0_2/1 -> Q_2/1
  D1_2/1 -> S0_2/2
  b0_2/1 -> S0_2/1
  S2_1/1 -> D2_1/1
  S1_1/1 -> D1_1/1
  na2_1/1 -> S2_1/2
  b2_1/1 -> S2_1/1
  D2_1/1 -> S1_1/3
  na1_1/1 -> S1_1/2
  b1_1/1 -> S1_1/1
  Q_1/1 -> b2_2/1, b1_2/1, b0_2/1, na2_1/1, na1_1/1
  S0_1/1 -> Q_1/1
  D1_1/1 -> S0_1/2
  b0_1/1 -> S0_1/1
  dataIn/1 -> b2_1/1, b1_1/1, b0_1/1
  validIn/1 -> validOut/1

== system HFMA_4B_1_5_9_13/Subsystem/HFMA1/Biquad Filter8 ==
  dataIn : Inport
  validIn : Inport  Port=2
  D1_1 : Delay  DelayLength=1  InitialCondition=0
  D1_2 : Delay  DelayLength=1  InitialCondition=0
  D2_1 : Delay  DelayLength=1  InitialCondition=0
  D2_2 : Delay  DelayLength=1  InitialCondition=0
  Q_1 : DataTypeConversion  OutDataTypeStr=fixdt(1,18,16)  RndMeth=Floor
  Q_2 : DataTypeConversion  OutDataTypeStr=fixdt(1,18,16)  RndMeth=Floor
  S0_1 : Sum  OutDataTypeStr=fixdt(1,40,30)  SaturateOnIntegerOverflow=on
  S0_2 : Sum  OutDataTypeStr=fixdt(1,40,30)  SaturateOnIntegerOverflow=on
  S1_1 : Sum  Inputs=+++  OutDataTypeStr=fixdt(1,40,30)  SaturateOnIntegerOverflow=on
  S1_2 : Sum  Inputs=+++  OutDataTypeStr=fixdt(1,40,30)  SaturateOnIntegerOverflow=on
  S2_1 : Sum  OutDataTypeStr=fixdt(1,40,30)  SaturateOnIntegerOverflow=on
  S2_2 : Sum  OutDataTypeStr=fixdt(1,40,30)  SaturateOnIntegerOverflow=on
  b0_1 : Gain  Gain=0.0011721199932606119  ParamDataTypeStr=fixdt(1,18,26)  OutDataTypeStr=fixdt(1,40,30)  SaturateOnIntegerOverflow=on
  b0_2 : Gain  Gain=0.0012157429617273841  ParamDataTypeStr=fixdt(1,18,26)  OutDataTypeStr=fixdt(1,40,30)  SaturateOnIntegerOverflow=on
  b1_1 : Gain  Gain=0.0023442399865212238  ParamDataTypeStr=fixdt(1,18,25)  OutDataTypeStr=fixdt(1,40,30)  SaturateOnIntegerOverflow=on
  b1_2 : Gain  Gain=0.0024314859234547681  ParamDataTypeStr=fixdt(1,18,25)  OutDataTypeStr=fixdt(1,40,30)  SaturateOnIntegerOverflow=on
  b2_1 : Gain  Gain=0.0011721199932606119  ParamDataTypeStr=fixdt(1,18,26)  OutDataTypeStr=fixdt(1,40,30)  SaturateOnIntegerOverflow=on
  b2_2 : Gain  Gain=0.0012157429617273841  ParamDataTypeStr=fixdt(1,18,26)  OutDataTypeStr=fixdt(1,40,30)  SaturateOnIntegerOverflow=on
  na1_1 : Gain  Gain=1.8728036090138058  ParamDataTypeStr=fixdt(1,18,16)  OutDataTypeStr=fixdt(1,40,30)  SaturateOnIntegerOverflow=on
  na1_2 : Gain  Gain=1.942504026420016  ParamDataTypeStr=fixdt(1,18,16)  OutDataTypeStr=fixdt(1,40,30)  SaturateOnIntegerOverflow=on
  na2_1 : Gain  Gain=-0.87749208898684827  ParamDataTypeStr=fixdt(1,18,17)  OutDataTypeStr=fixdt(1,40,30)  SaturateOnIntegerOverflow=on
  na2_2 : Gain  Gain=-0.9473669982669255  ParamDataTypeStr=fixdt(1,18,17)  OutDataTypeStr=fixdt(1,40,30)  SaturateOnIntegerOverflow=on
  dataOut : Outport
  validOut : Outport  Port=2
  wires:
  S2_2/1 -> D2_2/1
  S1_2/1 -> D1_2/1
  na2_2/1 -> S2_2/2
  b2_2/1 -> S2_2/1
  D2_2/1 -> S1_2/3
  na1_2/1 -> S1_2/2
  b1_2/1 -> S1_2/1
  Q_2/1 -> dataOut/1, na2_2/1, na1_2/1
  S0_2/1 -> Q_2/1
  D1_2/1 -> S0_2/2
  b0_2/1 -> S0_2/1
  S2_1/1 -> D2_1/1
  S1_1/1 -> D1_1/1
  na2_1/1 -> S2_1/2
  b2_1/1 -> S2_1/1
  D2_1/1 -> S1_1/3
  na1_1/1 -> S1_1/2
  b1_1/1 -> S1_1/1
  Q_1/1 -> b2_2/1, b1_2/1, b0_2/1, na2_1/1, na1_1/1
  S0_1/1 -> Q_1/1
  D1_1/1 -> S0_1/2
  b0_1/1 -> S0_1/1
  dataIn/1 -> b2_1/1, b1_1/1, b0_1/1
  validIn/1 -> validOut/1

== system HFMA_4B_1_5_9_13/Subsystem/HFMA1/Compare To Constant ==
  u : Inport
  Compare : RelationalOperator  Operator===  OutDataTypeStr=boolean
  Constant : Constant  DisableCoverage=on  Value=const  OutDataTypeStr=Inherit: Inherit via back propagation  SampleTime=-1
  y : Outport
  wires:
  Compare/1 -> y/1
  Constant/1 -> Compare/2
  u/1 -> Compare/1

== system HFMA_4B_1_5_9_13/Subsystem/HFMA1/Covariance Matrix ==
  X1_Re : Inport
  X1_Im : Inport  Port=2
  X2_Re : Inport  Port=3
  X2_Im : Inport  Port=4
  X3_Re : Inport  Port=5
  X3_Im : Inport  Port=6
  X4_Re : Inport  Port=7
  X4_Im : Inport  Port=8
  RESET : Inport  Port=9
  R1 : Subsystem
  R2 : Subsystem
  R21 : Subsystem
  R21_Re : Outport
  R21_Im : Outport  Port=2
  R31_Re : Outport  Port=3
  R31_Im : Outport  Port=4
  R41_Re : Outport  Port=5
  R41_Im : Outport  Port=6
  wires:
  X4_Re/1 -> R2/1(Xi_Re)
  X2_Re/1 -> R21/1(Xi_Re)
  R1/2(Rij_Im) -> R31_Im/1
  X3_Re/1 -> R1/1(Xi_Re)
  X1_Im/1 -> R2/4(Xj_Im), R1/4(Xj_Im), R21/4(Xj_Im)
  R21/1(Rij_Re) -> R21_Re/1
  X3_Im/1 -> R1/2(Xi_Im)
  R21/2(Rij_Im) -> R21_Im/1
  R1/1(Rij_Re) -> R31_Re/1
  X1_Re/1 -> R2/3(Xj_Re), R1/3(Xj_Re), R21/3(Xj_Re)
  RESET/1 -> R21/5(RESET), R2/5(RESET), R1/5(RESET)
  R2/2(Rij_Im) -> R41_Im/1
  X2_Im/1 -> R21/2(Xi_Im)
  R2/1(Rij_Re) -> R41_Re/1
  X4_Im/1 -> R2/2(Xi_Im)

== system HFMA_4B_1_5_9_13/Subsystem/HFMA1/Hardware Friendly MUSIC Algorithm ==
  R21_Re : Inport
  R21_Im : Inport  Port=2
  R31_Re : Inport  Port=3
  R31_Im : Inport  Port=4
  R41_Re : Inport  Port=5
  R41_Im : Inport  Port=6
  a1_Re : Inport  Port=7
  a1_Im : Inport  Port=8
  a2_Re : Inport  Port=9
  a2_Im : Inport  Port=10
  a3_Re : Inport  Port=11
  a3_Im : Inport  Port=12
  Add : Sum  Inputs=+++  OutDataTypeStr=fixdt(1,32,28)  SaturateOnIntegerOverflow=on
  Add1 : Sum  Inputs=+++  OutDataTypeStr=fixdt(1,32,28)  SaturateOnIntegerOverflow=on
  Add2 : Sum  OutDataTypeStr=fixdt(0,40,34)  SaturateOnIntegerOverflow=on
  Gain : Gain  Gain=-1  ParamDataTypeStr=fixdt(1,18,17)  OutDataTypeStr=fixdt(1,32,29)  SaturateOnIntegerOverflow=on
  Gain1 : Gain  Gain=-1  ParamDataTypeStr=fixdt(1,18,17)  OutDataTypeStr=fixdt(1,32,29)  SaturateOnIntegerOverflow=on
  Gain2 : Gain  Gain=-1  ParamDataTypeStr=fixdt(1,18,17)  OutDataTypeStr=fixdt(1,32,29)  SaturateOnIntegerOverflow=on
  Product : Product  OutDataTypeStr=fixdt(0,40,34)  SaturateOnIntegerOverflow=on
  Product1 : Product  OutDataTypeStr=fixdt(0,40,34)  SaturateOnIntegerOverflow=on
  complex multiplier1 : Subsystem
  complex multiplier2 : Subsystem
  complex multiplier3 : Subsystem
  P_Theta : Outport
  wires:
  Add1/1 -> Product1/1, Product1/2
  complex multiplier2/1(Re) -> Add/2
  a1_Re/1 -> complex multiplier1/3(u)
  R21_Im/1 -> Gain/1
  complex multiplier1/1(Re) -> Add/1
  complex multiplier1/2(Im) -> Add1/1
  Add2/1 -> P_Theta/1
  a2_Im/1 -> complex multiplier2/4(v)
  a3_Re/1 -> complex multiplier3/3(u)
  Product1/1 -> Add2/2
  Gain1/1 -> complex multiplier2/2(y)
  complex multiplier3/1(Re) -> Add/3
  Product/1 -> Add2/1
  a3_Im/1 -> complex multiplier3/4(v)
  Gain/1 -> complex multiplier1/2(y)
  R31_Im/1 -> Gain1/1
  complex multiplier2/2(Im) -> Add1/2
  R41_Im/1 -> Gain2/1
  Add/1 -> Product/2, Product/1
  R31_Re/1 -> complex multiplier2/1(x)
  a1_Im/1 -> complex multiplier1/4(v)
  R41_Re/1 -> complex multiplier3/1(x)
  a2_Re/1 -> complex multiplier2/3(u)
  complex multiplier3/2(Im) -> Add1/3
  Gain2/1 -> complex multiplier3/2(y)
  R21_Re/1 -> complex multiplier1/1(x)

== system HFMA_4B_1_5_9_13/Subsystem/HFMA1/I//Q Separation ==
  note: -2x[n]*sin((2*pi*f0*n)/fs)
  note: 2x[n]*cos((2*pi*f0*n)/fs)
  Microphone Input : Inport
  F0 Index : Inport  Port=2
  IQ Counter Input : Inport  Port=3
  Gain : Gain  Gain=-2  ParamDataTypeStr=fixdt(1,18,16)  OutDataTypeStr=fixdt(1,18,14)  SaturateOnIntegerOverflow=on
  Gain1 : Gain  Gain=2  ParamDataTypeStr=fixdt(0,18,16)  OutDataTypeStr=fixdt(1,18,14)  SaturateOnIntegerOverflow=on
  IdxConv{,1..3} (4 alike) : DataTypeConversion  OutDataTypeStr=uint8  RndMeth=Floor
  Product : Product  OutDataTypeStr=fixdt(1,18,15)  SaturateOnIntegerOverflow=on
  Product1 : Product  OutDataTypeStr=fixdt(1,18,15)  SaturateOnIntegerOverflow=on
  cosLUT : LookupNDDirect  Table=[cosLUT]  TableDataTypeStr=fixdt(1,18,16)
  sinLUT : LookupNDDirect  Table=[sinLUT]  TableDataTypeStr=fixdt(1,18,16)
  I[n] : Outport
  Q[n] : Outport  Port=2
  wires:
  Gain/1 -> Q[n]/1
  Gain1/1 -> I[n]/1
  Microphone Input/1 -> Product1/1, Product/1
  cosLUT/1 -> Product/2
  sinLUT/1 -> Product1/2
  Product/1 -> Gain1/1
  Product1/1 -> Gain/1
  F0 Index/1 -> IdxConv/1, IdxConv2/1
  IQ Counter Input/1 -> IdxConv1/1, IdxConv3/1
  IdxConv/1 -> cosLUT/1
  IdxConv1/1 -> cosLUT/2
  IdxConv2/1 -> sinLUT/1
  IdxConv3/1 -> sinLUT/2

== system HFMA_4B_1_5_9_13/Subsystem/HFMA1/I//Q Separation1 ==
  note: -2x[n]*sin((2*pi*f0*n)/fs)
  note: 2x[n]*cos((2*pi*f0*n)/fs)
  Microphone Input : Inport
  F0 Index : Inport  Port=2
  IQ Counter Input : Inport  Port=3
  Gain : Gain  Gain=-2  ParamDataTypeStr=fixdt(1,18,16)  OutDataTypeStr=fixdt(1,18,14)  SaturateOnIntegerOverflow=on
  Gain1 : Gain  Gain=2  ParamDataTypeStr=fixdt(0,18,16)  OutDataTypeStr=fixdt(1,18,14)  SaturateOnIntegerOverflow=on
  IdxConv{,1..3} (4 alike) : DataTypeConversion  OutDataTypeStr=uint8  RndMeth=Floor
  Product : Product  OutDataTypeStr=fixdt(1,18,15)  SaturateOnIntegerOverflow=on
  Product1 : Product  OutDataTypeStr=fixdt(1,18,15)  SaturateOnIntegerOverflow=on
  cosLUT : LookupNDDirect  Table=[cosLUT]  TableDataTypeStr=fixdt(1,18,16)
  sinLUT : LookupNDDirect  Table=[sinLUT]  TableDataTypeStr=fixdt(1,18,16)
  I[n] : Outport
  Q[n] : Outport  Port=2
  wires:
  Gain/1 -> Q[n]/1
  Gain1/1 -> I[n]/1
  Microphone Input/1 -> Product1/1, Product/1
  cosLUT/1 -> Product/2
  sinLUT/1 -> Product1/2
  Product/1 -> Gain1/1
  Product1/1 -> Gain/1
  F0 Index/1 -> IdxConv/1, IdxConv2/1
  IQ Counter Input/1 -> IdxConv1/1, IdxConv3/1
  IdxConv/1 -> cosLUT/1
  IdxConv1/1 -> cosLUT/2
  IdxConv2/1 -> sinLUT/1
  IdxConv3/1 -> sinLUT/2

== system HFMA_4B_1_5_9_13/Subsystem/HFMA1/I//Q Separation2 ==
  note: -2x[n]*sin((2*pi*f0*n)/fs)
  note: 2x[n]*cos((2*pi*f0*n)/fs)
  Microphone Input : Inport
  F0 Index : Inport  Port=2
  IQ Counter Input : Inport  Port=3
  Gain : Gain  Gain=-2  ParamDataTypeStr=fixdt(1,18,16)  OutDataTypeStr=fixdt(1,18,14)  SaturateOnIntegerOverflow=on
  Gain1 : Gain  Gain=2  ParamDataTypeStr=fixdt(0,18,16)  OutDataTypeStr=fixdt(1,18,14)  SaturateOnIntegerOverflow=on
  IdxConv{,1..3} (4 alike) : DataTypeConversion  OutDataTypeStr=uint8  RndMeth=Floor
  Product : Product  OutDataTypeStr=fixdt(1,18,15)  SaturateOnIntegerOverflow=on
  Product1 : Product  OutDataTypeStr=fixdt(1,18,15)  SaturateOnIntegerOverflow=on
  cosLUT : LookupNDDirect  Table=[cosLUT]  TableDataTypeStr=fixdt(1,18,16)
  sinLUT : LookupNDDirect  Table=[sinLUT]  TableDataTypeStr=fixdt(1,18,16)
  I[n] : Outport
  Q[n] : Outport  Port=2
  wires:
  Gain/1 -> Q[n]/1
  Gain1/1 -> I[n]/1
  Microphone Input/1 -> Product1/1, Product/1
  cosLUT/1 -> Product/2
  sinLUT/1 -> Product1/2
  Product/1 -> Gain1/1
  Product1/1 -> Gain/1
  F0 Index/1 -> IdxConv/1, IdxConv2/1
  IQ Counter Input/1 -> IdxConv1/1, IdxConv3/1
  IdxConv/1 -> cosLUT/1
  IdxConv1/1 -> cosLUT/2
  IdxConv2/1 -> sinLUT/1
  IdxConv3/1 -> sinLUT/2

== system HFMA_4B_1_5_9_13/Subsystem/HFMA1/I//Q Separation3 ==
  note: -2x[n]*sin((2*pi*f0*n)/fs)
  note: 2x[n]*cos((2*pi*f0*n)/fs)
  Microphone Input : Inport
  F0 Index : Inport  Port=2
  IQ Counter Input : Inport  Port=3
  Gain : Gain  Gain=-2  ParamDataTypeStr=fixdt(1,18,16)  OutDataTypeStr=fixdt(1,18,14)  SaturateOnIntegerOverflow=on
  Gain1 : Gain  Gain=2  ParamDataTypeStr=fixdt(0,18,16)  OutDataTypeStr=fixdt(1,18,14)  SaturateOnIntegerOverflow=on
  IdxConv{,1..3} (4 alike) : DataTypeConversion  OutDataTypeStr=uint8  RndMeth=Floor
  Product : Product  OutDataTypeStr=fixdt(1,18,15)  SaturateOnIntegerOverflow=on
  Product1 : Product  OutDataTypeStr=fixdt(1,18,15)  SaturateOnIntegerOverflow=on
  cosLUT : LookupNDDirect  Table=[cosLUT]  TableDataTypeStr=fixdt(1,18,16)
  sinLUT : LookupNDDirect  Table=[sinLUT]  TableDataTypeStr=fixdt(1,18,16)
  I[n] : Outport
  Q[n] : Outport  Port=2
  wires:
  Gain/1 -> Q[n]/1
  Gain1/1 -> I[n]/1
  Microphone Input/1 -> Product1/1, Product/1
  cosLUT/1 -> Product/2
  sinLUT/1 -> Product1/2
  Product/1 -> Gain1/1
  Product1/1 -> Gain/1
  F0 Index/1 -> IdxConv/1, IdxConv2/1
  IQ Counter Input/1 -> IdxConv1/1, IdxConv3/1
  IdxConv/1 -> cosLUT/1
  IdxConv1/1 -> cosLUT/2
  IdxConv2/1 -> sinLUT/1
  IdxConv3/1 -> sinLUT/2

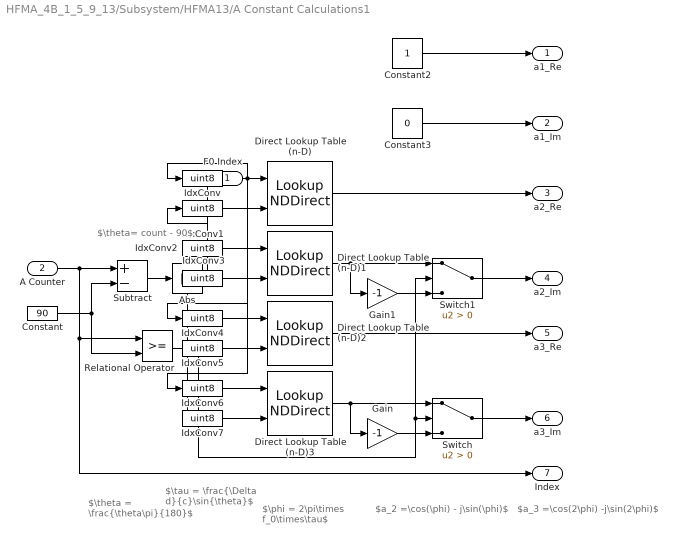
== system HFMA_4B_1_5_9_13/Subsystem/HFMA13/A Constant Calculations1 ==
  note: $\theta = \frac{\theta\pi}{180}$
  note: $\phi = 2\pi\times f_0\times\tau$
  note: $\tau = \frac{\Delta d}{c}\sin{\theta}$
  note: $\theta= count - 90$
  note: $a_2 =\cos(\phi) - j\sin(\phi)$
  note: $a_3 =\cos(2\phi) -j\sin(2\phi)$
  F0 Index : Inport
  A Counter : Inport  Port=2
  Abs : Abs  OutDataTypeStr=fixdt(1,18,0)  SaturateOnIntegerOverflow=off
  Constant : Constant  Value=90  OutDataTypeStr=fixdt(0,18,11)
  Constant2 : Constant  OutDataTypeStr=fixdt(0,18,17)
  Constant3 : Constant  Value=0  OutDataTypeStr=fixdt(1,18,4)
  Direct Lookup Table (n-D) : LookupNDDirect  Table=[a2_Re]  TableDataTypeStr=fixdt(1,18,16)
  Direct Lookup Table (n-D)1 : LookupNDDirect  Table=[a2_Im]  TableDataTypeStr=fixdt(1,18,16)
  Direct Lookup Table (n-D)2 : LookupNDDirect  Table=[a3_Re]  TableDataTypeStr=fixdt(1,18,16)
  Direct Lookup Table (n-D)3 : LookupNDDirect  Table=[a3_Im]  TableDataTypeStr=fixdt(1,18,16)
  Gain : Gain  Gain=-1  ParamDataTypeStr=fixdt(1,18,17)  OutDataTypeStr=fixdt(1,18,16)  SaturateOnIntegerOverflow=on
  Gain1 : Gain  Gain=-1  ParamDataTypeStr=fixdt(1,18,17)  OutDataTypeStr=fixdt(0,18,17)  SaturateOnIntegerOverflow=on
  IdxConv{,1..7} (8 alike) : DataTypeConversion  OutDataTypeStr=uint8  RndMeth=Floor
  Relational Operator : RelationalOperator  OutDataTypeStr=boolean  RndMeth=Simplest  InputSameDT=off
  Subtract : Sum  Inputs=+-  OutDataTypeStr=fixdt(1,18,0)  SaturateOnIntegerOverflow=on
  Switch : Switch  Criteria=u2 > Threshold  OutDataTypeStr=fixdt(1,18,16)  SaturateOnIntegerOverflow=off  InputSameDT=off
  Switch1 : Switch  Criteria=u2 > Threshold  OutDataTypeStr=fixdt(1,18,16)  SaturateOnIntegerOverflow=off  InputSameDT=off
  a1_Re : Outport
  a1_Im : Outport  Port=2
  a2_Re : Outport  Port=3
  a2_Im : Outport  Port=4
  a3_Re : Outport  Port=5
  a3_Im : Outport  Port=6
  Index : Outport  Port=7
  wires:
  A Counter/1 -> Relational Operator/1, Index/1, Subtract/1
  Constant/1 -> Subtract/2, Relational Operator/2
  Constant2/1 -> a1_Re/1
  Constant3/1 -> a1_Im/1
  F0 Index/1 -> IdxConv/1, IdxConv2/1, IdxConv4/1, IdxConv6/1
  Subtract/1 -> Abs/1
  Direct Lookup Table (n-D)/1 -> a2_Re/1
  Direct Lookup Table (n-D)2/1 -> a3_Re/1
  Direct Lookup Table (n-D)1/1 -> Switch1/1, Gain1/1
  Direct Lookup Table (n-D)3/1 -> Switch/1, Gain/1
  Gain/1 -> Switch/3
  Gain1/1 -> Switch1/3
  Relational Operator/1 -> Switch/2, Switch1/2
  Switch/1 -> a3_Im/1
  Switch1/1 -> a2_Im/1
  Abs/1 -> IdxConv1/1, IdxConv3/1, IdxConv5/1, IdxConv7/1
  IdxConv/1 -> Direct Lookup Table (n-D)/1
  IdxConv1/1 -> Direct Lookup Table (n-D)/2
  IdxConv2/1 -> Direct Lookup Table (n-D)1/1
  IdxConv3/1 -> Direct Lookup Table (n-D)1/2
  IdxConv4/1 -> Direct Lookup Table (n-D)2/1
  IdxConv5/1 -> Direct Lookup Table (n-D)2/2
  IdxConv6/1 -> Direct Lookup Table (n-D)3/1
  IdxConv7/1 -> Direct Lookup Table (n-D)3/2
